simulink model "nea_pidari_lv_feeder"  (R2024b)
settings: Solver=FixedStepDiscrete  StartTime=0.0  StopTime=0.2  FixedStep=2e-6  RelTol=1e-3
libraries: spsThreePhaseSeriesRLCBranchLib x9, spsThreePhaseVIMeasurementLib x9, spsThreePhaseParallelRLCLoadLib x8, spsThreePhaseSourceLib x1, spspowerguiLib x1
Description:
  | Pidari LV feeder: 100 kVA DT at Khajuri Chanha, 400 V
  | Loading 100 % of the FY 2082/83 recorded peak. PCC (for a prosumer connection) at A5 (PCC).
  | Built by matlab_models/build_nea_lv_feeder.m from nea_lv_feeder_data.m.
settings Model: Creator=subas  LastModifiedBy=subas

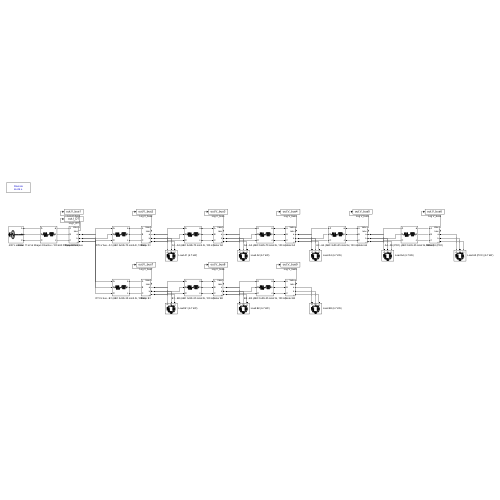
[thumbnail: Simulink's stored preview of the top-level diagram]
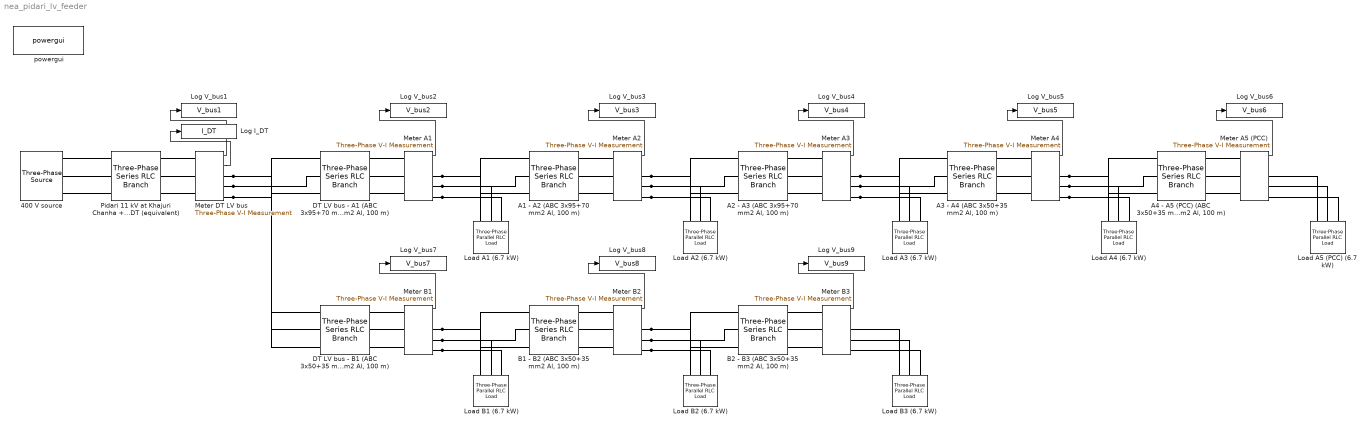
== system nea_pidari_lv_feeder ==
  400 V source : spsThreePhaseSourceLib/Three-Phase Source  InternalConnection=Yg  VoltagePhases=off  Voltage=350.1265303  PhaseAngle=0  Voltage_phases=[25e3 25e3 25e3]/sqrt(3)  PhaseAngles_phases=[0 -120 +120]  Frequency=50  NonIdealSource=off  SpecifyImpedance=off  Resistance=0.8929  Inductance=16.58e-3  ShortCircuitLevel=100e6  BaseVoltage=25e3  XRratio=7  BusType=swing  Pref=10e3  Qref=0  Prefabc=[10e3, 10e3, 10e3]  Qrefabc=[0, 0, 0]  Qmin=-inf  Qmax=inf
  "A1 - A2 (ABC 3x95+70 mm2 Al, 100 m)" : spsThreePhaseSeriesRLCBranchLib/Three-Phase Series RLC Branch  LConnTagsString=A|B|C  RConnTagsString=A|B|C  BranchType=RL  Resistance=0.0371584  Inductance=2.546479089e-05  Capacitance=1e-6  Measurements=None
  "A2 - A3 (ABC 3x95+70 mm2 Al, 100 m)" : spsThreePhaseSeriesRLCBranchLib/Three-Phase Series RLC Branch  LConnTagsString=A|B|C  RConnTagsString=A|B|C  BranchType=RL  Resistance=0.0371584  Inductance=2.546479089e-05  Capacitance=1e-6  Measurements=None
  "A3 - A4 (ABC 3x50+35 mm2 Al, 100 m)" : spsThreePhaseSeriesRLCBranchLib/Three-Phase Series RLC Branch  LConnTagsString=A|B|C  RConnTagsString=A|B|C  BranchType=RL  Resistance=0.07443292  Inductance=2.705634033e-05  Capacitance=1e-6  Measurements=None
  "A4 - A5 (PCC) (ABC 3x50+35 mm2 Al, 100 m)" : spsThreePhaseSeriesRLCBranchLib/Three-Phase Series RLC Branch  LConnTagsString=A|B|C  RConnTagsString=A|B|C  BranchType=RL  Resistance=0.07443292  Inductance=2.705634033e-05  Capacitance=1e-6  Measurements=None
  "B1 - B2 (ABC 3x50+35 mm2 Al, 100 m)" : spsThreePhaseSeriesRLCBranchLib/Three-Phase Series RLC Branch  LConnTagsString=A|B|C  RConnTagsString=A|B|C  BranchType=RL  Resistance=0.07443292  Inductance=2.705634033e-05  Capacitance=1e-6  Measurements=None
  "B2 - B3 (ABC 3x50+35 mm2 Al, 100 m)" : spsThreePhaseSeriesRLCBranchLib/Three-Phase Series RLC Branch  LConnTagsString=A|B|C  RConnTagsString=A|B|C  BranchType=RL  Resistance=0.07443292  Inductance=2.705634033e-05  Capacitance=1e-6  Measurements=None
  "DT LV bus - A1 (ABC 3x95+70 mm2 Al, 100 m)" : spsThreePhaseSeriesRLCBranchLib/Three-Phase Series RLC Branch  LConnTagsString=A|B|C  RConnTagsString=A|B|C  BranchType=RL  Resistance=0.0371584  Inductance=2.546479089e-05  Capacitance=1e-6  Measurements=None
  "DT LV bus - B1 (ABC 3x50+35 mm2 Al, 100 m)" : spsThreePhaseSeriesRLCBranchLib/Three-Phase Series RLC Branch  LConnTagsString=A|B|C  RConnTagsString=A|B|C  BranchType=RL  Resistance=0.07443292  Inductance=2.705634033e-05  Capacitance=1e-6  Measurements=None
  Load A1 (6.7 kW) : spsThreePhaseParallelRLCLoadLib/Three-Phase Parallel RLC Load  LConnTagsString=A|B|C  Configuration=Y (grounded)  NominalVoltage=400  Vabc=[1e3 1e3 1e3]  Vabcp=[1e3 1e3 1e3]  NominalFrequency=50  UnbalancedPower=off  ActivePower=9907.573187  InductivePower=6140.16239  CapacitivePower=0  Pabc=[10e3 9e3 11e3]  QLabc=[100 90 110]  QCabc=[100 90 110]  Pabcp=[10e3 9e3 11e3]  QLabcp=[100 90 110]  QCabcp=[100 90 110]  Measurements=None  LoadType=constant Z
  Load A2 (6.7 kW) : spsThreePhaseParallelRLCLoadLib/Three-Phase Parallel RLC Load  LConnTagsString=A|B|C  Configuration=Y (grounded)  NominalVoltage=400  Vabc=[1e3 1e3 1e3]  Vabcp=[1e3 1e3 1e3]  NominalFrequency=50  UnbalancedPower=off  ActivePower=10123.18189  InductivePower=6273.784663  CapacitivePower=0  Pabc=[10e3 9e3 11e3]  QLabc=[100 90 110]  QCabc=[100 90 110]  Pabcp=[10e3 9e3 11e3]  QLabcp=[100 90 110]  QCabcp=[100 90 110]  Measurements=None  LoadType=constant Z
  Load A3 (6.7 kW) : spsThreePhaseParallelRLCLoadLib/Three-Phase Parallel RLC Load  LConnTagsString=A|B|C  Configuration=Y (grounded)  NominalVoltage=400  Vabc=[1e3 1e3 1e3]  Vabcp=[1e3 1e3 1e3]  NominalFrequency=50  UnbalancedPower=off  ActivePower=10290.15735  InductivePower=6377.266758  CapacitivePower=0  Pabc=[10e3 9e3 11e3]  QLabc=[100 90 110]  QCabc=[100 90 110]  Pabcp=[10e3 9e3 11e3]  QLabcp=[100 90 110]  QCabcp=[100 90 110]  Measurements=None  LoadType=constant Z
  Load A4 (6.7 kW) : spsThreePhaseParallelRLCLoadLib/Three-Phase Parallel RLC Load  LConnTagsString=A|B|C  Configuration=Y (grounded)  NominalVoltage=400  Vabc=[1e3 1e3 1e3]  Vabcp=[1e3 1e3 1e3]  NominalFrequency=50  UnbalancedPower=off  ActivePower=10507.68303  InductivePower=6512.077065  CapacitivePower=0  Pabc=[10e3 9e3 11e3]  QLabc=[100 90 110]  QCabc=[100 90 110]  Pabcp=[10e3 9e3 11e3]  QLabcp=[100 90 110]  QCabcp=[100 90 110]  Measurements=None  LoadType=constant Z
  Load A5 (PCC) (6.7 kW) : spsThreePhaseParallelRLCLoadLib/Three-Phase Parallel RLC Load  LConnTagsString=A|B|C  Configuration=Y (grounded)  NominalVoltage=400  Vabc=[1e3 1e3 1e3]  Vabcp=[1e3 1e3 1e3]  NominalFrequency=50  UnbalancedPower=off  ActivePower=10619.20847  InductivePower=6581.194325  CapacitivePower=0  Pabc=[10e3 9e3 11e3]  QLabc=[100 90 110]  QCabc=[100 90 110]  Pabcp=[10e3 9e3 11e3]  QLabcp=[100 90 110]  QCabcp=[100 90 110]  Measurements=None  LoadType=constant Z
  Load B1 (6.7 kW) : spsThreePhaseParallelRLCLoadLib/Three-Phase Parallel RLC Load  LConnTagsString=A|B|C  Configuration=Y (grounded)  NominalVoltage=400  Vabc=[1e3 1e3 1e3]  Vabcp=[1e3 1e3 1e3]  NominalFrequency=50  UnbalancedPower=off  ActivePower=9940.874237  InductivePower=6160.800527  CapacitivePower=0  Pabc=[10e3 9e3 11e3]  QLabc=[100 90 110]  QCabc=[100 90 110]  Pabcp=[10e3 9e3 11e3]  QLabcp=[100 90 110]  QCabcp=[100 90 110]  Measurements=None  LoadType=constant Z
  Load B2 (6.7 kW) : spsThreePhaseParallelRLCLoadLib/Three-Phase Parallel RLC Load  LConnTagsString=A|B|C  Configuration=Y (grounded)  NominalVoltage=400  Vabc=[1e3 1e3 1e3]  Vabcp=[1e3 1e3 1e3]  NominalFrequency=50  UnbalancedPower=off  ActivePower=10143.6687  InductivePower=6286.481246  CapacitivePower=0  Pabc=[10e3 9e3 11e3]  QLabc=[100 90 110]  QCabc=[100 90 110]  Pabcp=[10e3 9e3 11e3]  QLabcp=[100 90 110]  QCabcp=[100 90 110]  Measurements=None  LoadType=constant Z
  Load B3 (6.7 kW) : spsThreePhaseParallelRLCLoadLib/Three-Phase Parallel RLC Load  LConnTagsString=A|B|C  Configuration=Y (grounded)  NominalVoltage=400  Vabc=[1e3 1e3 1e3]  Vabcp=[1e3 1e3 1e3]  NominalFrequency=50  UnbalancedPower=off  ActivePower=10247.55086  InductivePower=6350.861626  CapacitivePower=0  Pabc=[10e3 9e3 11e3]  QLabc=[100 90 110]  QCabc=[100 90 110]  Pabcp=[10e3 9e3 11e3]  QLabcp=[100 90 110]  QCabcp=[100 90 110]  Measurements=None  LoadType=constant Z
  Log I_DT : ToWorkspace  VariableName=I_DT  SaveFormat=Timeseries  SampleTime=-1
      settings: Decimation=10
  Log V_bus1 : ToWorkspace  VariableName=V_bus1  SaveFormat=Timeseries  SampleTime=-1
      settings: Decimation=10
  Log V_bus2 : ToWorkspace  VariableName=V_bus2  SaveFormat=Timeseries  SampleTime=-1
      settings: Decimation=10
  Log V_bus3 : ToWorkspace  VariableName=V_bus3  SaveFormat=Timeseries  SampleTime=-1
      settings: Decimation=10
  Log V_bus4 : ToWorkspace  VariableName=V_bus4  SaveFormat=Timeseries  SampleTime=-1
      settings: Decimation=10
  Log V_bus5 : ToWorkspace  VariableName=V_bus5  SaveFormat=Timeseries  SampleTime=-1
      settings: Decimation=10
  Log V_bus6 : ToWorkspace  VariableName=V_bus6  SaveFormat=Timeseries  SampleTime=-1
      settings: Decimation=10
  Log V_bus7 : ToWorkspace  VariableName=V_bus7  SaveFormat=Timeseries  SampleTime=-1
      settings: Decimation=10
  Log V_bus8 : ToWorkspace  VariableName=V_bus8  SaveFormat=Timeseries  SampleTime=-1
      settings: Decimation=10
  Log V_bus9 : ToWorkspace  VariableName=V_bus9  SaveFormat=Timeseries  SampleTime=-1
      settings: Decimation=10
  Meter A{1..4} (4 alike) : spsThreePhaseVIMeasurementLib/Three-Phase V-I Measurement  VoltageMeasurement=phase-to-ground  SetLabelV=off  LabelV=Vabc  Vpu=off  VpuLL=off  CurrentMeasurement=yes  SetLabelI=off  LabelI=Iabc  Ipu=off  Pbase=100e6  Vbase=500e3  OutputType=Complex  PhasorSimulation=off  PSBequivalent=0
  Meter A5 (PCC) : spsThreePhaseVIMeasurementLib/Three-Phase V-I Measurement  VoltageMeasurement=phase-to-ground  SetLabelV=off  LabelV=Vabc  Vpu=off  VpuLL=off  CurrentMeasurement=yes  SetLabelI=off  LabelI=Iabc  Ipu=off  Pbase=100e6  Vbase=500e3  OutputType=Complex  PhasorSimulation=off  PSBequivalent=0
  Meter B1 : spsThreePhaseVIMeasurementLib/Three-Phase V-I Measurement  VoltageMeasurement=phase-to-ground  SetLabelV=off  LabelV=Vabc  Vpu=off  VpuLL=off  CurrentMeasurement=yes  SetLabelI=off  LabelI=Iabc  Ipu=off  Pbase=100e6  Vbase=500e3  OutputType=Complex  PhasorSimulation=off  PSBequivalent=0
  Meter B2 : spsThreePhaseVIMeasurementLib/Three-Phase V-I Measurement  VoltageMeasurement=phase-to-ground  SetLabelV=off  LabelV=Vabc  Vpu=off  VpuLL=off  CurrentMeasurement=yes  SetLabelI=off  LabelI=Iabc  Ipu=off  Pbase=100e6  Vbase=500e3  OutputType=Complex  PhasorSimulation=off  PSBequivalent=0
  Meter B3 : spsThreePhaseVIMeasurementLib/Three-Phase V-I Measurement  VoltageMeasurement=phase-to-ground  SetLabelV=off  LabelV=Vabc  Vpu=off  VpuLL=off  CurrentMeasurement=yes  SetLabelI=off  LabelI=Iabc  Ipu=off  Pbase=100e6  Vbase=500e3  OutputType=Complex  PhasorSimulation=off  PSBequivalent=0
  Meter DT LV bus : spsThreePhaseVIMeasurementLib/Three-Phase V-I Measurement  VoltageMeasurement=phase-to-ground  SetLabelV=off  LabelV=Vabc  Vpu=off  VpuLL=off  CurrentMeasurement=yes  SetLabelI=off  LabelI=Iabc  Ipu=off  Pbase=100e6  Vbase=500e3  OutputType=Complex  PhasorSimulation=off  PSBequivalent=0
  Pidari 11 kV at Khajuri Chanha + 100 kVA DT (equivalent) : spsThreePhaseSeriesRLCBranchLib/Three-Phase Series RLC Branch  LConnTagsString=A|B|C  RConnTagsString=A|B|C  BranchType=RL  Resistance=0.05113738486  Inductance=0.0002982117468  Capacitance=1e-6  Measurements=None
  powergui : spspowerguiLib/powergui  Priority=1  SimulationMode=Discrete  SampleTime=2e-6  frequency=60  Iterations=50  frequencyindice=60  Pbase=100e6  ErrMax=1e-4  UnitsV=kV  UnitsW=MW  buscounter=0  FunctionMessages=off  echomessages=off  EnableUseOfTLC=off  CurrentSourceSwitches=off  DisableSnubberDevices=off  DisableRonSwitches=off  DisableVfSwitches=off  DisplayEquations=off  AutomaticDiscreteSolvers=off  SolverType=Tustin/Backward Euler (TBE)  Interpol=off  ExternalGateDelay=off  methode=off  Ts=100  x0status=blocks  SPID=on  SwTol=0  HookPort=off  NonlinearTolerance=1e-4  nMaxIteration=100  ContinueOnMaxIteration=off  RestoreLinks=warning  ResistiveCurrentMeasurement=off  Frange=[0:2:500]  Ylog=off  Xlog=on  ShowGrid=off  save=off  variable=ZData  structure=0  ZoomFFT=off  StartTime=0.0  cycles=1  DisplayStyle=1  fundamental=60  FreqAxis=off  MaxFrequency=1000  frequencyindicesteady=1  RmsSteady=1  display=off
  wires:
  Meter DT LV bus/1 -> Log V_bus1/1
  Meter DT LV bus/2 -> Log I_DT/1
  Meter A1/1 -> Log V_bus2/1
  Meter A2/1 -> Log V_bus3/1
  Meter A3/1 -> Log V_bus4/1
  Meter A4/1 -> Log V_bus5/1
  Meter A5 (PCC)/1 -> Log V_bus6/1
  Meter B1/1 -> Log V_bus7/1
  Meter B2/1 -> Log V_bus8/1
  Meter B3/1 -> Log V_bus9/1
  connections:
  400 V source/RConn1 -- Pidari 11 kV at Khajuri Chanha + 100 kVA DT (equivalent)/LConn1
  400 V source/RConn2 -- Pidari 11 kV at Khajuri Chanha + 100 kVA DT (equivalent)/LConn2
  400 V source/RConn3 -- Pidari 11 kV at Khajuri Chanha + 100 kVA DT (equivalent)/LConn3
  Pidari 11 kV at Khajuri Chanha + 100 kVA DT (equivalent)/RConn1 -- Meter DT LV bus/LConn1
  Pidari 11 kV at Khajuri Chanha + 100 kVA DT (equivalent)/RConn2 -- Meter DT LV bus/LConn2
  Pidari 11 kV at Khajuri Chanha + 100 kVA DT (equivalent)/RConn3 -- Meter DT LV bus/LConn3
  "DT LV bus - A1 (ABC 3x95+70 mm2 Al, 100 m)"/LConn1 -- Meter DT LV bus/RConn1 -- "DT LV bus - B1 (ABC 3x50+35 mm2 Al, 100 m)"/LConn1
  "DT LV bus - A1 (ABC 3x95+70 mm2 Al, 100 m)"/LConn2 -- Meter DT LV bus/RConn2 -- "DT LV bus - B1 (ABC 3x50+35 mm2 Al, 100 m)"/LConn2
  "DT LV bus - A1 (ABC 3x95+70 mm2 Al, 100 m)"/LConn3 -- Meter DT LV bus/RConn3 -- "DT LV bus - B1 (ABC 3x50+35 mm2 Al, 100 m)"/LConn3
  "DT LV bus - A1 (ABC 3x95+70 mm2 Al, 100 m)"/RConn1 -- Meter A1/LConn1
  "DT LV bus - A1 (ABC 3x95+70 mm2 Al, 100 m)"/RConn2 -- Meter A1/LConn2
  "DT LV bus - A1 (ABC 3x95+70 mm2 Al, 100 m)"/RConn3 -- Meter A1/LConn3
  "A1 - A2 (ABC 3x95+70 mm2 Al, 100 m)"/LConn1 -- Meter A1/RConn1 -- Load A1 (6.7 kW)/LConn1
  "A1 - A2 (ABC 3x95+70 mm2 Al, 100 m)"/LConn2 -- Meter A1/RConn2 -- Load A1 (6.7 kW)/LConn2
  "A1 - A2 (ABC 3x95+70 mm2 Al, 100 m)"/LConn3 -- Meter A1/RConn3 -- Load A1 (6.7 kW)/LConn3
  "A1 - A2 (ABC 3x95+70 mm2 Al, 100 m)"/RConn1 -- Meter A2/LConn1
  "A1 - A2 (ABC 3x95+70 mm2 Al, 100 m)"/RConn2 -- Meter A2/LConn2
  "A1 - A2 (ABC 3x95+70 mm2 Al, 100 m)"/RConn3 -- Meter A2/LConn3
  "A2 - A3 (ABC 3x95+70 mm2 Al, 100 m)"/LConn1 -- Meter A2/RConn1 -- Load A2 (6.7 kW)/LConn1
  "A2 - A3 (ABC 3x95+70 mm2 Al, 100 m)"/LConn2 -- Meter A2/RConn2 -- Load A2 (6.7 kW)/LConn2
  "A2 - A3 (ABC 3x95+70 mm2 Al, 100 m)"/LConn3 -- Meter A2/RConn3 -- Load A2 (6.7 kW)/LConn3
  "A2 - A3 (ABC 3x95+70 mm2 Al, 100 m)"/RConn1 -- Meter A3/LConn1
  "A2 - A3 (ABC 3x95+70 mm2 Al, 100 m)"/RConn2 -- Meter A3/LConn2
  "A2 - A3 (ABC 3x95+70 mm2 Al, 100 m)"/RConn3 -- Meter A3/LConn3
  "A3 - A4 (ABC 3x50+35 mm2 Al, 100 m)"/LConn1 -- Meter A3/RConn1 -- Load A3 (6.7 kW)/LConn1
  "A3 - A4 (ABC 3x50+35 mm2 Al, 100 m)"/LConn2 -- Meter A3/RConn2 -- Load A3 (6.7 kW)/LConn2
  "A3 - A4 (ABC 3x50+35 mm2 Al, 100 m)"/LConn3 -- Meter A3/RConn3 -- Load A3 (6.7 kW)/LConn3
  "A3 - A4 (ABC 3x50+35 mm2 Al, 100 m)"/RConn1 -- Meter A4/LConn1
  "A3 - A4 (ABC 3x50+35 mm2 Al, 100 m)"/RConn2 -- Meter A4/LConn2
  "A3 - A4 (ABC 3x50+35 mm2 Al, 100 m)"/RConn3 -- Meter A4/LConn3
  "A4 - A5 (PCC) (ABC 3x50+35 mm2 Al, 100 m)"/LConn1 -- Meter A4/RConn1 -- Load A4 (6.7 kW)/LConn1
  "A4 - A5 (PCC) (ABC 3x50+35 mm2 Al, 100 m)"/LConn2 -- Meter A4/RConn2 -- Load A4 (6.7 kW)/LConn2
  "A4 - A5 (PCC) (ABC 3x50+35 mm2 Al, 100 m)"/LConn3 -- Meter A4/RConn3 -- Load A4 (6.7 kW)/LConn3
  "A4 - A5 (PCC) (ABC 3x50+35 mm2 Al, 100 m)"/RConn1 -- Meter A5 (PCC)/LConn1
  "A4 - A5 (PCC) (ABC 3x50+35 mm2 Al, 100 m)"/RConn2 -- Meter A5 (PCC)/LConn2
  "A4 - A5 (PCC) (ABC 3x50+35 mm2 Al, 100 m)"/RConn3 -- Meter A5 (PCC)/LConn3
  "DT LV bus - B1 (ABC 3x50+35 mm2 Al, 100 m)"/RConn1 -- Meter B1/LConn1
  "DT LV bus - B1 (ABC 3x50+35 mm2 Al, 100 m)"/RConn2 -- Meter B1/LConn2
  "DT LV bus - B1 (ABC 3x50+35 mm2 Al, 100 m)"/RConn3 -- Meter B1/LConn3
  "B1 - B2 (ABC 3x50+35 mm2 Al, 100 m)"/LConn1 -- Meter B1/RConn1 -- Load B1 (6.7 kW)/LConn1
  "B1 - B2 (ABC 3x50+35 mm2 Al, 100 m)"/LConn2 -- Meter B1/RConn2 -- Load B1 (6.7 kW)/LConn2
  "B1 - B2 (ABC 3x50+35 mm2 Al, 100 m)"/LConn3 -- Meter B1/RConn3 -- Load B1 (6.7 kW)/LConn3
  "B1 - B2 (ABC 3x50+35 mm2 Al, 100 m)"/RConn1 -- Meter B2/LConn1
  "B1 - B2 (ABC 3x50+35 mm2 Al, 100 m)"/RConn2 -- Meter B2/LConn2
  "B1 - B2 (ABC 3x50+35 mm2 Al, 100 m)"/RConn3 -- Meter B2/LConn3
  "B2 - B3 (ABC 3x50+35 mm2 Al, 100 m)"/LConn1 -- Meter B2/RConn1 -- Load B2 (6.7 kW)/LConn1
  "B2 - B3 (ABC 3x50+35 mm2 Al, 100 m)"/LConn2 -- Meter B2/RConn2 -- Load B2 (6.7 kW)/LConn2
  "B2 - B3 (ABC 3x50+35 mm2 Al, 100 m)"/LConn3 -- Meter B2/RConn3 -- Load B2 (6.7 kW)/LConn3
  "B2 - B3 (ABC 3x50+35 mm2 Al, 100 m)"/RConn1 -- Meter B3/LConn1
  "B2 - B3 (ABC 3x50+35 mm2 Al, 100 m)"/RConn2 -- Meter B3/LConn2
  "B2 - B3 (ABC 3x50+35 mm2 Al, 100 m)"/RConn3 -- Meter B3/LConn3
  Meter A5 (PCC)/RConn1 -- Load A5 (PCC) (6.7 kW)/LConn1
  Meter A5 (PCC)/RConn2 -- Load A5 (PCC) (6.7 kW)/LConn2
  Meter A5 (PCC)/RConn3 -- Load A5 (PCC) (6.7 kW)/LConn3
  Meter B3/RConn1 -- Load B3 (6.7 kW)/LConn1
  Meter B3/RConn2 -- Load B3 (6.7 kW)/LConn2
  Meter B3/RConn3 -- Load B3 (6.7 kW)/LConn3
